simulink model "Bazen_DC_Ohrev_500m3_SK"  (R2026a)
settings: Solver=ode4  StopTime=604800  FixedStep=60
settings Model: Creator=Lysda  LastModifiedBy=Lysda

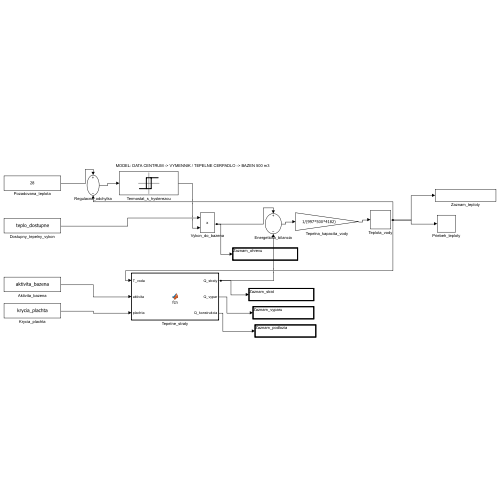
[thumbnail: Simulink's stored preview of the top-level diagram]
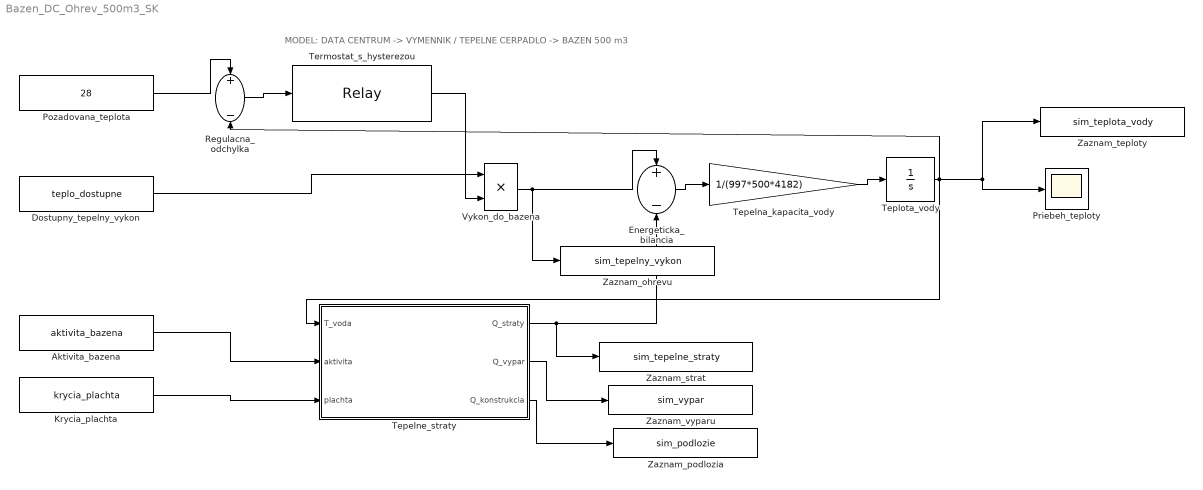
== system Bazen_DC_Ohrev_500m3_SK ==
  note: MODEL: DATA CENTRUM -> VYMENNIK / TEPELNE CERPADLO -> BAZEN 500 m3
  Aktivita_bazena : FromWorkspace  VariableName=aktivita_bazena
  Dostupny_tepelny_vykon : FromWorkspace  VariableName=teplo_dostupne
  Energeticka_bilancia : Sum  Inputs=+-
  Krycia_plachta : FromWorkspace  VariableName=krycia_plachta
  Pozadovana_teplota : Constant  Value=28
  Priebeh_teploty : Scope
  Regulacna_odchylka : Sum  Inputs=+-
  Tepelna_kapacita_vody : Gain  Gain=1/(997*500*4182)
  Tepelne_straty : MATLAB Function  TreatAsAtomicUnit=on
  Teplota_vody : Integrator  InitialCondition=16
  Termostat_s_hysterezou : Relay  OnSwitchValue=0.2  OffSwitchValue=-0.2
  Vykon_do_bazena : Product  Inputs=**
  Zaznam_ohrevu : ToWorkspace  VariableName=sim_tepelny_vykon  SaveFormat=Timeseries  SampleTime=-1
  Zaznam_podlozia : ToWorkspace  VariableName=sim_podlozie  SaveFormat=Timeseries  SampleTime=-1
  Zaznam_strat : ToWorkspace  VariableName=sim_tepelne_straty  SaveFormat=Timeseries  SampleTime=-1
  Zaznam_teploty : ToWorkspace  VariableName=sim_teplota_vody  SaveFormat=Timeseries  SampleTime=-1
  Zaznam_vyparu : ToWorkspace  VariableName=sim_vypar  SaveFormat=Timeseries  SampleTime=-1
  wires:
  Pozadovana_teplota/1 -> Regulacna_odchylka/1
  Teplota_vody/1 -> Zaznam_teploty/1, Priebeh_teploty/1, Regulacna_odchylka/2, Tepelne_straty/1(T_voda)
  Regulacna_odchylka/1 -> Termostat_s_hysterezou/1
  Dostupny_tepelny_vykon/1 -> Vykon_do_bazena/1
  Termostat_s_hysterezou/1 -> Vykon_do_bazena/2
  Vykon_do_bazena/1 -> Energeticka_bilancia/1, Zaznam_ohrevu/1
  Aktivita_bazena/1 -> Tepelne_straty/2(aktivita)
  Krycia_plachta/1 -> Tepelne_straty/3(plachta)
  Tepelne_straty/1(Q_straty) -> Energeticka_bilancia/2, Zaznam_strat/1
  Energeticka_bilancia/1 -> Tepelna_kapacita_vody/1
  Tepelna_kapacita_vody/1 -> Teplota_vody/1
  Tepelne_straty/2(Q_vypar) -> Zaznam_vyparu/1
  Tepelne_straty/3(Q_konstrukcia) -> Zaznam_podlozia/1

== matlab function Bazen_DC_Ohrev_500m3_SK/Tepelne_straty ==
  data: T_voda input; Q_straty output; aktivita input; plachta input; Q_vypar output; Q_konstrukcia output
function [Q_straty,Q_vypar,Q_konstrukcia] = strata(T_voda,aktivita,plachta)


%#codegen


% Fyzikalne rovnice, jednotky: W, degC, kg/s, Pa/kPa.


A=312.5; h=3; UA=800; cp=4182;


pvoda=0.61094*exp(17.625*T_voda/(T_voda+243.04));


pvzduch=0.60*0.61094*exp(17.625*29/(29+243.04));


mvypar=max(0,4e-5*A*(pvoda-pvzduch)*aktivita*(1-0.90*plachta));


Q_vypar=mvypar*2440000;


Q_konv=3*A*(T_voda-29)*(1-0.75*plachta);


Q_rad=0.95*5.670374419e-8*A*((T_voda+273.15)^4-(27+273.15)^4)*(1-0.75*plachta);


Q_konstrukcia=UA*(T_voda-20);


Q_doplnanie=mvypar*cp*(T_voda-15);


Q_straty=Q_vypar+Q_konv+Q_rad+Q_konstrukcia+Q_doplnanie+2000;


end
